simulink model "ACC4_FFNN_trainoss_30_30_30_ep_100_Nor_20250528"  (R2021a)
settings: Solver=FixedStepAuto  StartTime=0.0  StopTime=T  RelTol=1e-3
undefined symbols (not defined in the file or in its folder): t_gap, Ts, v0_ego, v0_lead, v_set, x0_ego, x0_lead, x_gain, x_offset, y_gain, y_offset
libraries: neural x95
(part 1 of 5)
settings Model: Creator=The MathWorks, Inc.  LastModifiedBy=deyun
settings SolverCC: AlgebraicLoopSolver=TrustRegion
settings DataIOCC: ReturnWorkspaceOutputs=off
settings DebuggingCC: ArithmeticOperatorsInVariantConditions=warning
settings SFSimCC: SimUseLocalCustomCode=off  CustomCodeUndefinedFunction=UseInterfaceOnly
settings RTWCC: RTWUseLocalCustomCode=off
settings CodeAppCC: StateflowObjectComments=on

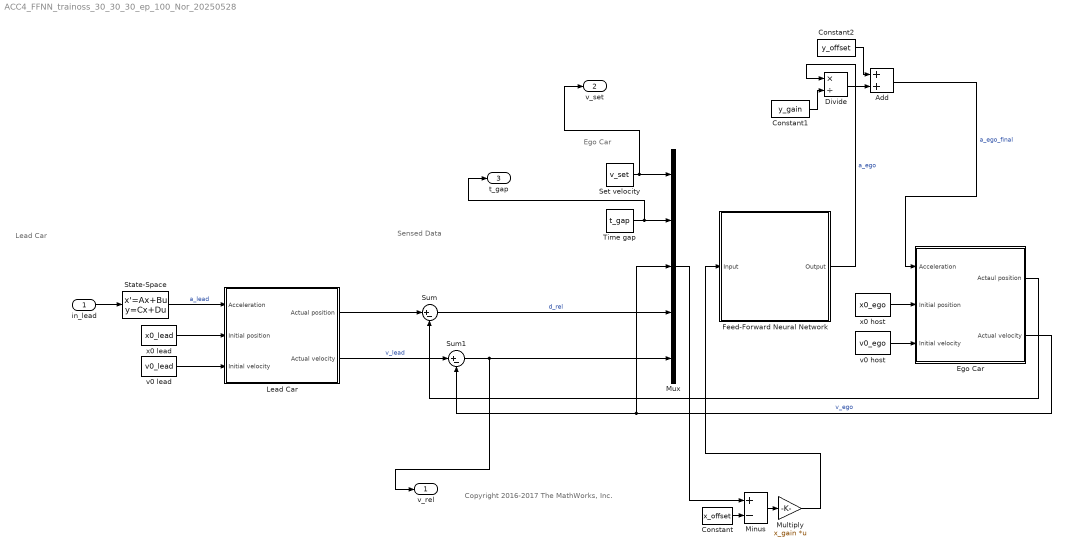
== system ACC4_FFNN_trainoss_30_30_30_ep_100_Nor_20250528 ==
  note: Sensed Data
  note: Lead Car
  note: Ego Car
  note: Copyright 2016-2017 The MathWorks, Inc.
  in_lead : Inport
  Add : Sum
  Constant : Constant  Value=x_offset
  Constant1 : Constant  Value=y_gain
  Constant2 : Constant  Value=y_offset
  Divide : Product  Inputs=*/
  Ego Car : Subsystem
  Feed-Forward Neural Network : Subsystem
      mask help: Feed-Forward Neural Network
      mask Display: e = 0.06;c1 = [120 150 230]/255;c2 = ([120 150 230]+0)/383;c3 = ([120 150 230]+128)/383;patch([0 1 1 0],[0 0 1 1],c1);patch([0 1 1 1-e 1-e 0+e],[0 0 1 1-e 0+e 0+e],c2);patch([0 0 1 1-e 0+e 0+e],[0 1 1 1-e 1-e 0+e],c3);plot([0 1 1 0 0],[0 0 1 1 0]);fprintf('NNET');port_label('input',1,' Input');port_label('output',1,'Output ');
  Lead Car : Subsystem
  Minus : Sum  Inputs=+-
  Multiply : Gain  Gain=x_gain  Multiplication=Matrix(K*u)
  Mux : Mux  Inputs=5
  Set velocity : Constant  Value=v_set  SampleTime=Ts
  State-Space : StateSpace  A=-10  B=10  D=0  InitialCondition=0
  Sum : Sum  Inputs=|+-
  Sum1 : Sum  Inputs=|+-
  Time gap : Constant  Value=t_gap  SampleTime=Ts
  v0 host : Constant  Value=v0_ego  SampleTime=Ts
  v0 lead : Constant  Value=v0_lead  SampleTime=Ts
  x0 host : Constant  Value=x0_ego  SampleTime=Ts
  x0 lead : Constant  Value=x0_lead  SampleTime=Ts
  v_rel : Outport
  v_set : Outport  Port=2
  t_gap : Outport  Port=3
  wires:
  x0 lead/1 -> Lead Car/2(Initial position)
  v0 lead/1 -> Lead Car/3(Initial velocity)
  x0 host/1 -> Ego Car/2(Initial position)
  Ego Car/1(Actaul position) -> Sum/2
  Ego Car/2(Actual velocity) -> Mux/3, Sum1/2  "v_ego"
  v0 host/1 -> Ego Car/3(Initial velocity)
  Set velocity/1 -> v_set/1, Mux/1
  Feed-Forward Neural Network/1(Output) -> Divide/1  "a_ego"
  Lead Car/1(Actual position) -> Sum/1
  Sum1/1 -> v_rel/1, Mux/5
  State-Space/1 -> Lead Car/1(Acceleration)  "a_lead"
  Lead Car/2(Actual velocity) -> Sum1/1  "v_lead"
  Sum/1 -> Mux/4  "d_rel"
  in_lead/1 -> State-Space/1
  Time gap/1 -> t_gap/1, Mux/2
  Mux/1 -> Minus/1
  Minus/1 -> Multiply/1
  Constant/1 -> Minus/2
  Multiply/1 -> Feed-Forward Neural Network/1(Input)
  Constant1/1 -> Divide/2
  Divide/1 -> Add/2
  Constant2/1 -> Add/1
  Add/1 -> Ego Car/1(Acceleration)  "a_ego_final"

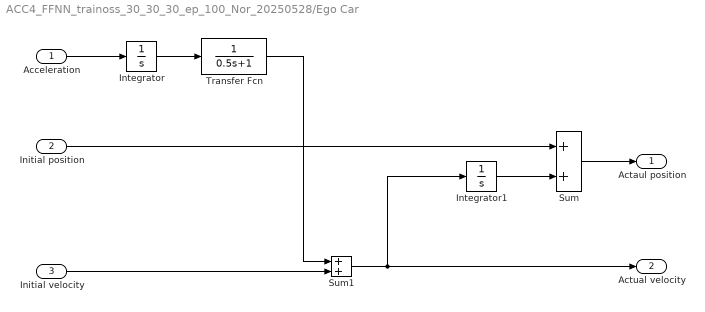
== system ACC4_FFNN_trainoss_30_30_30_ep_100_Nor_20250528/Ego Car ==
  Acceleration : Inport
  Initial position : Inport  Port=2
  Initial velocity : Inport  Port=3
  Integrator : Integrator
  Integrator1 : Integrator
  Sum : Sum
  Sum1 : Sum
  Transfer Fcn : TransferFcn  Denominator=[0.5 1]
  Actaul position : Outport  VectorParamsAs1DForOutWhenUnconnected=off
  Actual velocity : Outport  Port=2  VectorParamsAs1DForOutWhenUnconnected=off
  wires:
  Sum1/1 -> Integrator1/1, Actual velocity/1
  Initial velocity/1 -> Sum1/2
  Sum/1 -> Actaul position/1
  Transfer Fcn/1 -> Sum1/1
  Integrator/1 -> Transfer Fcn/1
  Acceleration/1 -> Integrator/1
  Initial position/1 -> Sum/1
  Integrator1/1 -> Sum/2

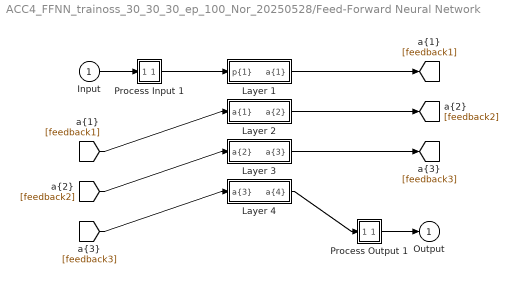
== system ACC4_FFNN_trainoss_30_30_30_ep_100_Nor_20250528/Feed-Forward Neural Network ==
  Input : Inport  PortDimensions=5
      mask Display: e = 0.06;c1 = [120 230 180]/255;c2 = ([120 230 180]+0)/(256+128);c3 = ([120 230 180]+128)/(256+128);patch([0 1 1 0],[0 0 1 1],c1);patch([0 1 1 1-e 1-e 0+e],[0 0 1 1-e 0+e 0+e],c2);patch([0 0 1 1-e 0+e 0+e],[0 1 1 1-e 1-e 0+e],c3);plot([0 1 1 0 0],[0 0 1 1 0]);
  Layer 1 : Subsystem
      mask Display: e = 0.06;c1 = [120 150 230]/255;c2 = ([120 150 230]+0)/383;c3 = ([120 150 230]+128)/383;patch([0 1 1 0],[0 0 1 1],c1);patch([0 1 1 1-e 1-e 0+e],[0 0 1 1-e 0+e 0+e],c2);patch([0 0 1 1-e 0+e 0+e],[0 1 1 1-e 1-e 0+e],c3);plot([0 1 1 0 0],[0 0 1 1 0]);
  Layer 2 : Subsystem
      mask Display: e = 0.06;c1 = [120 150 230]/255;c2 = ([120 150 230]+0)/383;c3 = ([120 150 230]+128)/383;patch([0 1 1 0],[0 0 1 1],c1);patch([0 1 1 1-e 1-e 0+e],[0 0 1 1-e 0+e 0+e],c2);patch([0 0 1 1-e 0+e 0+e],[0 1 1 1-e 1-e 0+e],c3);plot([0 1 1 0 0],[0 0 1 1 0]);
  Layer 3 : Subsystem
      mask Display: e = 0.06;c1 = [120 150 230]/255;c2 = ([120 150 230]+0)/383;c3 = ([120 150 230]+128)/383;patch([0 1 1 0],[0 0 1 1],c1);patch([0 1 1 1-e 1-e 0+e],[0 0 1 1-e 0+e 0+e],c2);patch([0 0 1 1-e 0+e 0+e],[0 1 1 1-e 1-e 0+e],c3);plot([0 1 1 0 0],[0 0 1 1 0]);
  Layer 4 : Subsystem
      mask Display: e = 0.06;c1 = [120 150 230]/255;c2 = ([120 150 230]+0)/383;c3 = ([120 150 230]+128)/383;patch([0 1 1 0],[0 0 1 1],c1);patch([0 1 1 1-e 1-e 0+e],[0 0 1 1-e 0+e 0+e],c2);patch([0 0 1 1-e 0+e 0+e],[0 1 1 1-e 1-e 0+e],c3);plot([0 1 1 0 0],[0 0 1 1 0]);
  Process Input 1 : Subsystem
      mask Display: e = 0.06;c1 = [120 150 230]/255;c2 = ([120 150 230]+0)/383;c3 = ([120 150 230]+128)/383;patch([0 1 1 0],[0 0 1 1],c1);patch([0 1 1 1-e 1-e 0+e],[0 0 1 1-e 0+e 0+e],c2);patch([0 0 1 1-e 0+e 0+e],[0 1 1 1-e 1-e 0+e],c3);plot([0 1 1 0 0],[0 0 1 1 0]);
  Process Output 1 : Subsystem
      mask Display: e = 0.06;c1 = [120 150 230]/255;c2 = ([120 150 230]+0)/383;c3 = ([120 150 230]+128)/383;patch([0 1 1 0],[0 0 1 1],c1);patch([0 1 1 1-e 1-e 0+e],[0 0 1 1-e 0+e 0+e],c2);patch([0 0 1 1-e 0+e 0+e],[0 1 1 1-e 1-e 0+e],c3);plot([0 1 1 0 0],[0 0 1 1 0]);
  Output : Outport  InitialOutput=0
      mask Display: e = 0.06;c1 = [120 230 180]/255;c2 = ([120 230 180]+0)/(256+128);c3 = ([120 230 180]+128)/(256+128);patch([0 1 1 0],[0 0 1 1],c1);patch([0 1 1 1-e 1-e 0+e],[0 0 1 1-e 0+e 0+e],c2);patch([0 0 1 1-e 0+e 0+e],[0 1 1 1-e 1-e 0+e],c3);plot([0 1 1 0 0],[0 0 1 1 0]);
  wires:
  Layer 4/1("a{4}") -> Process Output 1/1(a)
  [feedback3] -> Layer 4/1("a{3} ")
  Layer 3/1("a{3}") -> [feedback3]
  [feedback2] -> Layer 3/1("a{2} ")
  Layer 2/1("a{2}") -> [feedback2]
  [feedback1] -> Layer 2/1("a{1} ")
  Layer 1/1("a{1}") -> [feedback1]
  Process Input 1/1(p) -> Layer 1/1("p{1}")
  Process Output 1/1(y) -> Output/1
  Input/1 -> Process Input 1/1(x)

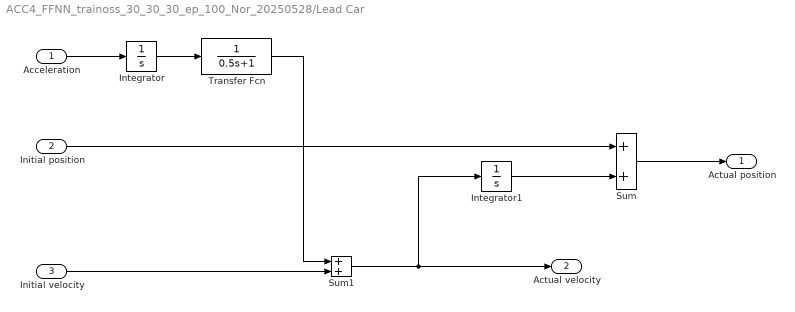
== system ACC4_FFNN_trainoss_30_30_30_ep_100_Nor_20250528/Lead Car ==
  Acceleration : Inport
  Initial position : Inport  Port=2
  Initial velocity : Inport  Port=3
  Integrator : Integrator
  Integrator1 : Integrator
  Sum : Sum
  Sum1 : Sum
  Transfer Fcn : TransferFcn  Denominator=[0.5 1]
  Actual position : Outport  VectorParamsAs1DForOutWhenUnconnected=off
  Actual velocity : Outport  Port=2  VectorParamsAs1DForOutWhenUnconnected=off
  wires:
  Transfer Fcn/1 -> Sum1/1
  Initial velocity/1 -> Sum1/2
  Sum/1 -> Actual position/1
  Integrator/1 -> Transfer Fcn/1
  Sum1/1 -> Integrator1/1, Actual velocity/1
  Acceleration/1 -> Integrator/1
  Initial position/1 -> Sum/1
  Integrator1/1 -> Sum/2

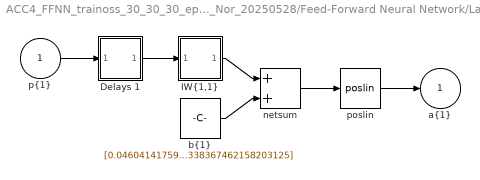
== system ACC4_FFNN_trainoss_30_30_30_ep_100_Nor_20250528/Feed-Forward Neural Network/Layer 1 ==
  "p{1}" : Inport  PortDimensions=5
      mask Display: e = 0.06;c1 = [120 230 180]/255;c2 = ([120 230 180]+0)/(256+128);c3 = ([120 230 180]+128)/(256+128);patch([0 1 1 0],[0 0 1 1],c1);patch([0 1 1 1-e 1-e 0+e],[0 0 1 1-e 0+e 0+e],c2);patch([0 0 1 1-e 0+e 0+e],[0 1 1 1-e 1-e 0+e],c3);plot([0 1 1 0 0],[0 0 1 1 0]);
  Delays 1 : Subsystem
      mask Display: e = 0.06;c1 = [120 150 230]/255;c2 = ([120 150 230]+0)/383;c3 = ([120 150 230]+128)/383;patch([0 1 1 0],[0 0 1 1],c1);patch([0 1 1 1-e 1-e 0+e],[0 0 1 1-e 0+e 0+e],c2);patch([0 0 1 1-e 0+e 0+e],[0 1 1 1-e 1-e 0+e],c3);plot([0 1 1 0 0],[0 0 1 1 0]);disp('0');
  "IW{1,1}" : Subsystem
      mask Display: e = 0.06;c1 = [120 150 230]/255;c2 = ([120 150 230]+0)/383;c3 = ([120 150 230]+128)/383;patch([0 1 1 0],[0 0 1 1],c1);patch([0 1 1 1-e 1-e 0+e],[0 0 1 1-e 0+e 0+e],c2);patch([0 0 1 1-e 0+e 0+e],[0 1 1 1-e 1-e 0+e],c3);plot([0 1 1 0 0],[0 0 1 1 0]);disp('W');
  "b{1}" : Constant  Value=[0.04604141759447825943407650584049406461417675018310546875;-0.349402015011147870637842061114497482776641845703125;0.667080116762796659912737595732323825359344482421875;0.60557904669735662661622654923121444880962371826171875;0.1282078326952769964375278277657344006001949310302734375;-0.4740719325396856032028836125391535460948944091796875;0.3611324046089003925175120457424782216548919677734375;-0.5341019862836020593022112734615802764892578125;-0.087117774565917793783142997199320234358310699462890625;-0.230866210976952146438634372316300868988037109375;0.077202877396043589897089987061917781829833984375;1.0034549741499108055364786196150816977024078369140625;0.50277941477063325947938210447318851947784423828125;0.955691922098945934038738414528779685497283935546875;-0.497741463247540483205710870606708340346813201904296875;0.04250082924725286093181608748636790551245212554931640625;-0.897127892866184328823919713613577187061309814453125;0.5137509419692445344907127946498803794384002685546875;0.20395953255102039491930554504506289958953857421875;0.70482076515493818913427048755693249404430389404296875;0.95254607457197948416904864643584005534648895263671875;0.8512508612841169775009575459989719092845916748046875;-0.1655257909270722027628153227851726114749908447265625;-1.001197592605171049484624745673500001430511474609375;0.08635824799345669100514299998394562862813472747802734375;-0.5845387560078811883812477390165440738201141357421875;-0.5614328236351393552894251115503720939159393310546875;-0.35187840556543503733877287231734953820705413818359375;-0.80810116678483101537722177454270422458648681640625;0.4950673234766060915035268408246338367462158203125]
      mask Display: e = 0.06;c1 = [120 150 230]/255;c2 = ([120 150 230]+0)/383;c3 = ([120 150 230]+128)/383;patch([0 1 1 0],[0 0 1 1],c1);patch([0 1 1 1-e 1-e 0+e],[0 0 1 1-e 0+e 0+e],c2);patch([0 0 1 1-e 0+e 0+e],[0 1 1 1-e 1-e 0+e],c3);plot([0 1 1 0 0],[0 0 1 1 0]);disp('b');
  netsum : Sum  Inputs=2  InputSameDT=on  SaturateOnIntegerOverflow=on  OutDataTypeStr=Inherit: Same as first input
      mask Display: e = 0.06;c1 = [120 150 230]/255;c2 = ([120 150 230]+0)/383;c3 = ([120 150 230]+128)/383;patch([0 1 1 0],[0 0 1 1],c1);patch([0 1 1 1-e 1-e 0+e],[0 0 1 1-e 0+e 0+e],c2);patch([0 0 1 1-e 0+e 0+e],[0 1 1 1-e 1-e 0+e],c3);plot([0 1 1 0 0],[0 0 1 1 0]);disp('+');
  poslin : neural/Transfer Functions/poslin
      settings: SourceProductBaseCode=NN
  "a{1}" : Outport  InitialOutput=[0;0;0;0;0;0;0;0;0;0;0;0;0;0;0;0;0;0;0;0;0;0;0;0;0;0;0;0;0;0]
      mask Display: e = 0.06;c1 = [120 230 180]/255;c2 = ([120 230 180]+0)/(256+128);c3 = ([120 230 180]+128)/(256+128);patch([0 1 1 0],[0 0 1 1],c1);patch([0 1 1 1-e 1-e 0+e],[0 0 1 1-e 0+e 0+e],c2);patch([0 0 1 1-e 0+e 0+e],[0 1 1 1-e 1-e 0+e],c3);plot([0 1 1 0 0],[0 0 1 1 0]);
  wires:
  poslin/1 -> "a{1}"/1
  netsum/1 -> poslin/1
  "b{1}"/1 -> netsum/2
  "IW{1,1}"/1("iz{1,1}") -> netsum/1
  Delays 1/1("pd{1,1}") -> "IW{1,1}"/1("pd{1,1}")
  "p{1}"/1 -> Delays 1/1("p{1}")

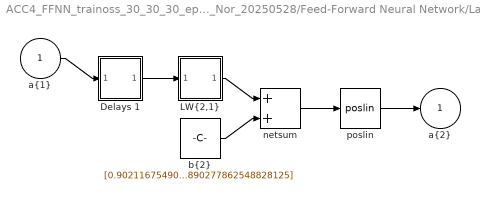
== system ACC4_FFNN_trainoss_30_30_30_ep_100_Nor_20250528/Feed-Forward Neural Network/Layer 2 ==
  "a{1} " : Inport  PortDimensions=30
      mask Display: e = 0.06;c1 = [120 230 180]/255;c2 = ([120 230 180]+0)/(256+128);c3 = ([120 230 180]+128)/(256+128);patch([0 1 1 0],[0 0 1 1],c1);patch([0 1 1 1-e 1-e 0+e],[0 0 1 1-e 0+e 0+e],c2);patch([0 0 1 1-e 0+e 0+e],[0 1 1 1-e 1-e 0+e],c3);plot([0 1 1 0 0],[0 0 1 1 0]);
  Delays 1 : Subsystem
      mask Display: e = 0.06;c1 = [120 150 230]/255;c2 = ([120 150 230]+0)/383;c3 = ([120 150 230]+128)/383;patch([0 1 1 0],[0 0 1 1],c1);patch([0 1 1 1-e 1-e 0+e],[0 0 1 1-e 0+e 0+e],c2);patch([0 0 1 1-e 0+e 0+e],[0 1 1 1-e 1-e 0+e],c3);plot([0 1 1 0 0],[0 0 1 1 0]);disp('0');
  "LW{2,1}" : Subsystem
      mask Display: e = 0.06;c1 = [120 150 230]/255;c2 = ([120 150 230]+0)/383;c3 = ([120 150 230]+128)/383;patch([0 1 1 0],[0 0 1 1],c1);patch([0 1 1 1-e 1-e 0+e],[0 0 1 1-e 0+e 0+e],c2);patch([0 0 1 1-e 0+e 0+e],[0 1 1 1-e 1-e 0+e],c3);plot([0 1 1 0 0],[0 0 1 1 0]);disp('W');
  "b{2}" : Constant  Value=[0.90211675490508869135197755895205773413181304931640625;0.96364395097861355043988851321046240627765655517578125;-0.93801236425877643210213818747433833777904510498046875;-0.01526552283014774580305328299800748936831951141357421875;0.725444256277659516030098529881797730922698974609375;-0.51151540170335441093385497879353351891040802001953125;0.66538113127496512078096202458254992961883544921875;0.6269149410732415272917705806321464478969573974609375;0.258930692402123241446787460517953149974346160888671875;-0.99391093407740893628243838975322432816028594970703125;-0.2405521205461311762263676428119651973247528076171875;0.8088428445387572107705409507616423070430755615234375;0.364640259893649842926066639847704209387302398681640625;-0.243645218450386613628921850249753333628177642822265625;0.2639094214046682207452931834268383681774139404296875;-0.5134609550588200566068053376511670649051666259765625;0.1373606272949773610125845380025566555559635162353515625;0.97668827905990884818976383030530996620655059814453125;0.69526590032446000666510599330649711191654205322265625;-0.434971195316202818847983735395246185362339019775390625;0.364915328900436097825377146364189684391021728515625;-0.279865051883634141649537241391954012215137481689453125;0.97740122180252420047708028505439870059490203857421875;-0.832027408487622466282118693925440311431884765625;-0.49423259242849260086671847602701745927333831787109375;0.626024890630703101379594954778440296649932861328125;-0.8310643492461855519337632358656264841556549072265625;0.0627983927541861941534762081573717296123504638671875;0.601245958295900440049308599554933607578277587890625;0.477951473350415156904347213639994151890277862548828125]
      mask Display: e = 0.06;c1 = [120 150 230]/255;c2 = ([120 150 230]+0)/383;c3 = ([120 150 230]+128)/383;patch([0 1 1 0],[0 0 1 1],c1);patch([0 1 1 1-e 1-e 0+e],[0 0 1 1-e 0+e 0+e],c2);patch([0 0 1 1-e 0+e 0+e],[0 1 1 1-e 1-e 0+e],c3);plot([0 1 1 0 0],[0 0 1 1 0]);disp('b');
  netsum : Sum  Inputs=2  InputSameDT=on  SaturateOnIntegerOverflow=on  OutDataTypeStr=Inherit: Same as first input
      mask Display: e = 0.06;c1 = [120 150 230]/255;c2 = ([120 150 230]+0)/383;c3 = ([120 150 230]+128)/383;patch([0 1 1 0],[0 0 1 1],c1);patch([0 1 1 1-e 1-e 0+e],[0 0 1 1-e 0+e 0+e],c2);patch([0 0 1 1-e 0+e 0+e],[0 1 1 1-e 1-e 0+e],c3);plot([0 1 1 0 0],[0 0 1 1 0]);disp('+');
  poslin : neural/Transfer Functions/poslin
      settings: SourceProductBaseCode=NN
  "a{2}" : Outport  InitialOutput=[0;0;0;0;0;0;0;0;0;0;0;0;0;0;0;0;0;0;0;0;0;0;0;0;0;0;0;0;0;0]
      mask Display: e = 0.06;c1 = [120 230 180]/255;c2 = ([120 230 180]+0)/(256+128);c3 = ([120 230 180]+128)/(256+128);patch([0 1 1 0],[0 0 1 1],c1);patch([0 1 1 1-e 1-e 0+e],[0 0 1 1-e 0+e 0+e],c2);patch([0 0 1 1-e 0+e 0+e],[0 1 1 1-e 1-e 0+e],c3);plot([0 1 1 0 0],[0 0 1 1 0]);
  wires:
  poslin/1 -> "a{2}"/1
  netsum/1 -> poslin/1
  "b{2}"/1 -> netsum/2
  "LW{2,1}"/1("lz{2,1}") -> netsum/1
  Delays 1/1("pd{2,1}") -> "LW{2,1}"/1("ad{2,1}")
  "a{1} "/1 -> Delays 1/1("p{2}")

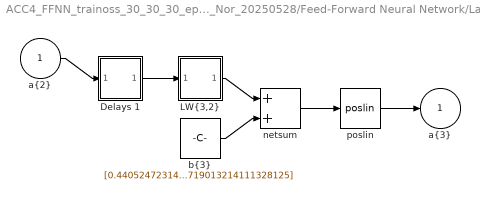
== system ACC4_FFNN_trainoss_30_30_30_ep_100_Nor_20250528/Feed-Forward Neural Network/Layer 3 ==
  "a{2} " : Inport  PortDimensions=30
      mask Display: e = 0.06;c1 = [120 230 180]/255;c2 = ([120 230 180]+0)/(256+128);c3 = ([120 230 180]+128)/(256+128);patch([0 1 1 0],[0 0 1 1],c1);patch([0 1 1 1-e 1-e 0+e],[0 0 1 1-e 0+e 0+e],c2);patch([0 0 1 1-e 0+e 0+e],[0 1 1 1-e 1-e 0+e],c3);plot([0 1 1 0 0],[0 0 1 1 0]);
  Delays 1 : Subsystem
      mask Display: e = 0.06;c1 = [120 150 230]/255;c2 = ([120 150 230]+0)/383;c3 = ([120 150 230]+128)/383;patch([0 1 1 0],[0 0 1 1],c1);patch([0 1 1 1-e 1-e 0+e],[0 0 1 1-e 0+e 0+e],c2);patch([0 0 1 1-e 0+e 0+e],[0 1 1 1-e 1-e 0+e],c3);plot([0 1 1 0 0],[0 0 1 1 0]);disp('0');
  "LW{3,2}" : Subsystem
      mask Display: e = 0.06;c1 = [120 150 230]/255;c2 = ([120 150 230]+0)/383;c3 = ([120 150 230]+128)/383;patch([0 1 1 0],[0 0 1 1],c1);patch([0 1 1 1-e 1-e 0+e],[0 0 1 1-e 0+e 0+e],c2);patch([0 0 1 1-e 0+e 0+e],[0 1 1 1-e 1-e 0+e],c3);plot([0 1 1 0 0],[0 0 1 1 0]);disp('W');
  "b{3}" : Constant  Value=[0.4405247231410467367851424569380469620227813720703125;0.357876687390491110551948850115877576172351837158203125;-0.574481979793593833250042735016904771327972412109375;-0.837153308541852769764091135584749281406402587890625;-0.45146469146650824999511542046093381941318511962890625;0.73604643553605664241246131496154703199863433837890625;0.11830618425636067747586110954216565005481243133544921875;-0.0710728139228912481062394590480835177004337310791015625;-0.1393981984391927664290733446250669658184051513671875;0.54797184004082755137687854585237801074981689453125;0.308241831903243002077630308122024871408939361572265625;0.31545304820107766818892969240550883114337921142578125;-0.67808294548384340227897837394266389310359954833984375;-0.135258081328783585917108212015591561794281005859375;0.010172168711043649835801261360757052898406982421875;-0.25362159832491959488010024870163761079311370849609375;-0.039723153024012018696975445664065773598849773406982421875;-0.31521694315790338425387062670779414474964141845703125;0.55514550915098548333759254092001356184482574462890625;-0.2321122752203861328013090314925648272037506103515625;0.42332375192715809841814689207240007817745208740234375;-0.040123747740405980855005196872298256494104862213134765625;0.45836044424314348333382440614514052867889404296875;0.8749288536162034279897170563344843685626983642578125;0.034051484090962598483276480010317754931747913360595703125;0.80611753338239744426374500108067877590656280517578125;-0.56333564819738002338311844141571782529354095458984375;0.746490829761710994461054724524728953838348388671875;-0.8343950519130831633418665660428814589977264404296875;-0.06910200297563613702767071345078875310719013214111328125]
      mask Display: e = 0.06;c1 = [120 150 230]/255;c2 = ([120 150 230]+0)/383;c3 = ([120 150 230]+128)/383;patch([0 1 1 0],[0 0 1 1],c1);patch([0 1 1 1-e 1-e 0+e],[0 0 1 1-e 0+e 0+e],c2);patch([0 0 1 1-e 0+e 0+e],[0 1 1 1-e 1-e 0+e],c3);plot([0 1 1 0 0],[0 0 1 1 0]);disp('b');
  netsum : Sum  Inputs=2  InputSameDT=on  SaturateOnIntegerOverflow=on  OutDataTypeStr=Inherit: Same as first input
      mask Display: e = 0.06;c1 = [120 150 230]/255;c2 = ([120 150 230]+0)/383;c3 = ([120 150 230]+128)/383;patch([0 1 1 0],[0 0 1 1],c1);patch([0 1 1 1-e 1-e 0+e],[0 0 1 1-e 0+e 0+e],c2);patch([0 0 1 1-e 0+e 0+e],[0 1 1 1-e 1-e 0+e],c3);plot([0 1 1 0 0],[0 0 1 1 0]);disp('+');
  poslin : neural/Transfer Functions/poslin
      settings: SourceProductBaseCode=NN
  "a{3}" : Outport  InitialOutput=[0;0;0;0;0;0;0;0;0;0;0;0;0;0;0;0;0;0;0;0;0;0;0;0;0;0;0;0;0;0]
      mask Display: e = 0.06;c1 = [120 230 180]/255;c2 = ([120 230 180]+0)/(256+128);c3 = ([120 230 180]+128)/(256+128);patch([0 1 1 0],[0 0 1 1],c1);patch([0 1 1 1-e 1-e 0+e],[0 0 1 1-e 0+e 0+e],c2);patch([0 0 1 1-e 0+e 0+e],[0 1 1 1-e 1-e 0+e],c3);plot([0 1 1 0 0],[0 0 1 1 0]);
  wires:
  poslin/1 -> "a{3}"/1
  netsum/1 -> poslin/1
  "b{3}"/1 -> netsum/2
  "LW{3,2}"/1("lz{3,2}") -> netsum/1
  Delays 1/1("pd{3,2}") -> "LW{3,2}"/1("ad{3,2}")
  "a{2} "/1 -> Delays 1/1("p{3}")

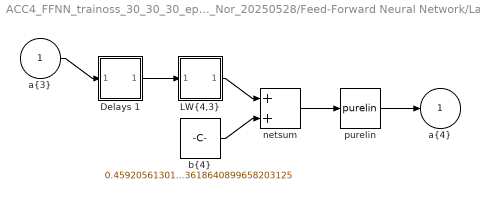
== system ACC4_FFNN_trainoss_30_30_30_ep_100_Nor_20250528/Feed-Forward Neural Network/Layer 4 ==
  "a{3} " : Inport  PortDimensions=30
      mask Display: e = 0.06;c1 = [120 230 180]/255;c2 = ([120 230 180]+0)/(256+128);c3 = ([120 230 180]+128)/(256+128);patch([0 1 1 0],[0 0 1 1],c1);patch([0 1 1 1-e 1-e 0+e],[0 0 1 1-e 0+e 0+e],c2);patch([0 0 1 1-e 0+e 0+e],[0 1 1 1-e 1-e 0+e],c3);plot([0 1 1 0 0],[0 0 1 1 0]);
  Delays 1 : Subsystem
      mask Display: e = 0.06;c1 = [120 150 230]/255;c2 = ([120 150 230]+0)/383;c3 = ([120 150 230]+128)/383;patch([0 1 1 0],[0 0 1 1],c1);patch([0 1 1 1-e 1-e 0+e],[0 0 1 1-e 0+e 0+e],c2);patch([0 0 1 1-e 0+e 0+e],[0 1 1 1-e 1-e 0+e],c3);plot([0 1 1 0 0],[0 0 1 1 0]);disp('0');
  "LW{4,3}" : Subsystem
      mask Display: e = 0.06;c1 = [120 150 230]/255;c2 = ([120 150 230]+0)/383;c3 = ([120 150 230]+128)/383;patch([0 1 1 0],[0 0 1 1],c1);patch([0 1 1 1-e 1-e 0+e],[0 0 1 1-e 0+e 0+e],c2);patch([0 0 1 1-e 0+e 0+e],[0 1 1 1-e 1-e 0+e],c3);plot([0 1 1 0 0],[0 0 1 1 0]);disp('W');
  "b{4}" : Constant  Value=0.459205613013363933561095109325833618640899658203125
      mask Display: e = 0.06;c1 = [120 150 230]/255;c2 = ([120 150 230]+0)/383;c3 = ([120 150 230]+128)/383;patch([0 1 1 0],[0 0 1 1],c1);patch([0 1 1 1-e 1-e 0+e],[0 0 1 1-e 0+e 0+e],c2);patch([0 0 1 1-e 0+e 0+e],[0 1 1 1-e 1-e 0+e],c3);plot([0 1 1 0 0],[0 0 1 1 0]);disp('b');
  netsum : Sum  Inputs=2  InputSameDT=on  SaturateOnIntegerOverflow=on  OutDataTypeStr=Inherit: Same as first input
      mask Display: e = 0.06;c1 = [120 150 230]/255;c2 = ([120 150 230]+0)/383;c3 = ([120 150 230]+128)/383;patch([0 1 1 0],[0 0 1 1],c1);patch([0 1 1 1-e 1-e 0+e],[0 0 1 1-e 0+e 0+e],c2);patch([0 0 1 1-e 0+e 0+e],[0 1 1 1-e 1-e 0+e],c3);plot([0 1 1 0 0],[0 0 1 1 0]);disp('+');
  purelin : neural/Transfer Functions/purelin
  "a{4}" : Outport  InitialOutput=0
      mask Display: e = 0.06;c1 = [120 230 180]/255;c2 = ([120 230 180]+0)/(256+128);c3 = ([120 230 180]+128)/(256+128);patch([0 1 1 0],[0 0 1 1],c1);patch([0 1 1 1-e 1-e 0+e],[0 0 1 1-e 0+e 0+e],c2);patch([0 0 1 1-e 0+e 0+e],[0 1 1 1-e 1-e 0+e],c3);plot([0 1 1 0 0],[0 0 1 1 0]);
  wires:
  purelin/1 -> "a{4}"/1
  netsum/1 -> purelin/1
  "b{4}"/1 -> netsum/2
  "LW{4,3}"/1("lz{4,3}") -> netsum/1
  Delays 1/1("pd{4,3}") -> "LW{4,3}"/1("ad{4,3}")
  "a{3} "/1 -> Delays 1/1("p{4}")

== system ACC4_FFNN_trainoss_30_30_30_ep_100_Nor_20250528/Feed-Forward Neural Network/Process Input 1 ==
  x : Inport  PortDimensions=5
      mask Display: e = 0.06;c1 = [120 230 180]/255;c2 = ([120 230 180]+0)/(256+128);c3 = ([120 230 180]+128)/(256+128);patch([0 1 1 0],[0 0 1 1],c1);patch([0 1 1 1-e 1-e 0+e],[0 0 1 1-e 0+e 0+e],c2);patch([0 0 1 1-e 0+e 0+e],[0 1 1 1-e 1-e 0+e],c3);plot([0 1 1 0 0],[0 0 1 1 0]);
  p : Outport  PortDimensions=5
      mask Display: e = 0.06;c1 = [120 230 180]/255;c2 = ([120 230 180]+0)/(256+128);c3 = ([120 230 180]+128)/(256+128);patch([0 1 1 0],[0 0 1 1],c1);patch([0 1 1 1-e 1-e 0+e],[0 0 1 1-e 0+e 0+e],c2);patch([0 0 1 1-e 0+e 0+e],[0 1 1 1-e 1-e 0+e],c3);plot([0 1 1 0 0],[0 0 1 1 0]);
  wires:
  x/1 -> p/1

== system ACC4_FFNN_trainoss_30_30_30_ep_100_Nor_20250528/Feed-Forward Neural Network/Process Output 1 ==
  a : Inport  PortDimensions=1
      mask Display: e = 0.06;c1 = [120 230 180]/255;c2 = ([120 230 180]+0)/(256+128);c3 = ([120 230 180]+128)/(256+128);patch([0 1 1 0],[0 0 1 1],c1);patch([0 1 1 1-e 1-e 0+e],[0 0 1 1-e 0+e 0+e],c2);patch([0 0 1 1-e 0+e 0+e],[0 1 1 1-e 1-e 0+e],c3);plot([0 1 1 0 0],[0 0 1 1 0]);
  y : Outport  PortDimensions=1
      mask Display: e = 0.06;c1 = [120 230 180]/255;c2 = ([120 230 180]+0)/(256+128);c3 = ([120 230 180]+128)/(256+128);patch([0 1 1 0],[0 0 1 1],c1);patch([0 1 1 1-e 1-e 0+e],[0 0 1 1-e 0+e 0+e],c2);patch([0 0 1 1-e 0+e 0+e],[0 1 1 1-e 1-e 0+e],c3);plot([0 1 1 0 0],[0 0 1 1 0]);
  wires:
  a/1 -> y/1

== system ACC4_FFNN_trainoss_30_30_30_ep_100_Nor_20250528/Feed-Forward Neural Network/Layer 1/Delays 1 ==
  "p{1}" : Inport  PortDimensions=5
      mask Display: e = 0.06;c1 = [120 230 180]/255;c2 = ([120 230 180]+0)/(256+128);c3 = ([120 230 180]+128)/(256+128);patch([0 1 1 0],[0 0 1 1],c1);patch([0 1 1 1-e 1-e 0+e],[0 0 1 1-e 0+e 0+e],c2);patch([0 0 1 1-e 0+e 0+e],[0 1 1 1-e 1-e 0+e],c3);plot([0 1 1 0 0],[0 0 1 1 0]);
  mux : Mux  Inputs=1
      mask Display: e = 0.06;c1 = [120 150 230]/255;c2 = ([120 150 230]+0)/383;c3 = ([120 150 230]+128)/383;patch([0 1 1 0],[0 0 1 1],c1);patch([0 1 1 1-e 1-e 0+e],[0 0 1 1-e 0+e 0+e],c2);patch([0 0 1 1-e 0+e 0+e],[0 1 1 1-e 1-e 0+e],c3);plot([0 1 1 0 0],[0 0 1 1 0]);disp('Mux')
  "pd{1,1}" : Outport
      mask Display: e = 0.06;c1 = [120 230 180]/255;c2 = ([120 230 180]+0)/(256+128);c3 = ([120 230 180]+128)/(256+128);patch([0 1 1 0],[0 0 1 1],c1);patch([0 1 1 1-e 1-e 0+e],[0 0 1 1-e 0+e 0+e],c2);patch([0 0 1 1-e 0+e 0+e],[0 1 1 1-e 1-e 0+e],c3);plot([0 1 1 0 0],[0 0 1 1 0]);
  wires:
  mux/1 -> "pd{1,1}"/1
  "p{1}"/1 -> mux/1

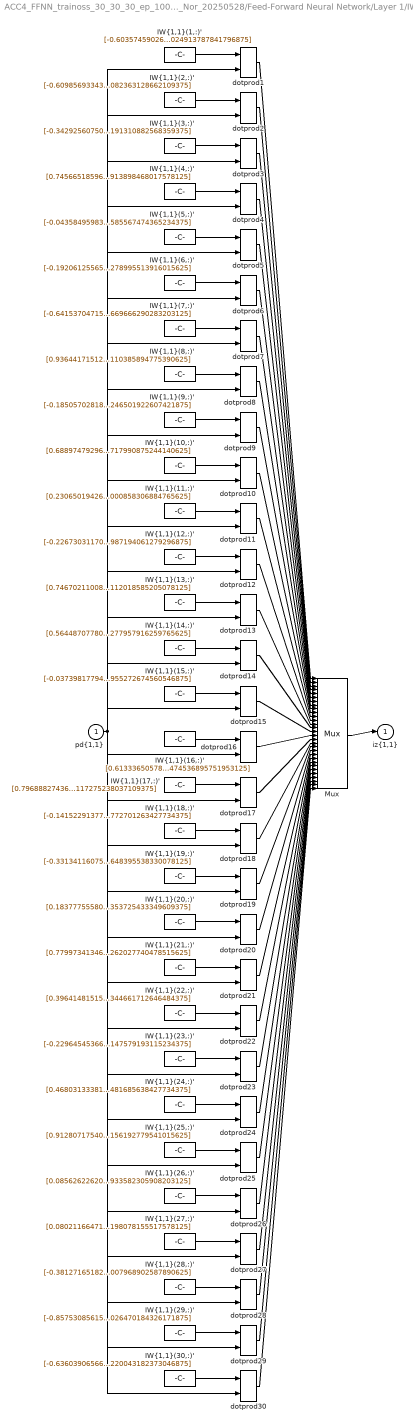
== system ACC4_FFNN_trainoss_30_30_30_ep_100_Nor_20250528/Feed-Forward Neural Network/Layer 1/IW{1,1} ==
  "pd{1,1}" : Inport  PortDimensions=5
      mask Display: e = 0.06;c1 = [120 230 180]/255;c2 = ([120 230 180]+0)/(256+128);c3 = ([120 230 180]+128)/(256+128);patch([0 1 1 0],[0 0 1 1],c1);patch([0 1 1 1-e 1-e 0+e],[0 0 1 1-e 0+e 0+e],c2);patch([0 0 1 1-e 0+e 0+e],[0 1 1 1-e 1-e 0+e],c3);plot([0 1 1 0 0],[0 0 1 1 0]);
  "IW{1,1}(1,:)'" : Constant  Value=[-0.6035745902618299130182322187465615570545196533203125;-0.814040325548151866286161748575977981090545654296875;-0.0775546564559805029492878247765474952757358551025390625;0.713774809937765208900373181677423417568206787109375;0.7908289690471679289629491904634051024913787841796875]
      mask Display: e = 0.06;c1 = [120 150 230]/255;c2 = ([120 150 230]+0)/383;c3 = ([120 150 230]+128)/383;patch([0 1 1 0],[0 0 1 1],c1);patch([0 1 1 1-e 1-e 0+e],[0 0 1 1-e 0+e 0+e],c2);patch([0 0 1 1-e 0+e 0+e],[0 1 1 1-e 1-e 0+e],c3);plot([0 1 1 0 0],[0 0 1 1 0]);disp('Weights');
  "IW{1,1}(10,:)'" : Constant  Value=[0.6889747929668963433158523912425152957439422607421875;-0.745467933349733158365779672749340534210205078125;-0.64204969474453577049644081853330135345458984375;0.799965592865721664139755375799722969532012939453125;-0.6903424584977886357961551766493357717990875244140625]
      mask Display: e = 0.06;c1 = [120 150 230]/255;c2 = ([120 150 230]+0)/383;c3 = ([120 150 230]+128)/383;patch([0 1 1 0],[0 0 1 1],c1);patch([0 1 1 1-e 1-e 0+e],[0 0 1 1-e 0+e 0+e],c2);patch([0 0 1 1-e 0+e 0+e],[0 1 1 1-e 1-e 0+e],c3);plot([0 1 1 0 0],[0 0 1 1 0]);disp('Weights');
  "IW{1,1}(11,:)'" : Constant  Value=[0.230650194261698970876750536262989044189453125;-0.982704624243819324647120083682239055633544921875;0.2666671606402430949600557141820900142192840576171875;-0.6131324961218160840559221469447948038578033447265625;-0.71218334265026417284616400138475000858306884765625]
      mask Display: e = 0.06;c1 = [120 150 230]/255;c2 = ([120 150 230]+0)/383;c3 = ([120 150 230]+128)/383;patch([0 1 1 0],[0 0 1 1],c1);patch([0 1 1 1-e 1-e 0+e],[0 0 1 1-e 0+e 0+e],c2);patch([0 0 1 1-e 0+e 0+e],[0 1 1 1-e 1-e 0+e],c3);plot([0 1 1 0 0],[0 0 1 1 0]);disp('Weights');
  "IW{1,1}(12,:)'" : Constant  Value=[-0.2267303117085231745075901699237874709069728851318359375;0.474206734523056783192629382028826512396335601806640625;0.26408373958160080707813222034019418060779571533203125;0.500370970455730645909397935611195862293243408203125;0.2109635849565252019299776975458371452987194061279296875]
      mask Display: e = 0.06;c1 = [120 150 230]/255;c2 = ([120 150 230]+0)/383;c3 = ([120 150 230]+128)/383;patch([0 1 1 0],[0 0 1 1],c1);patch([0 1 1 1-e 1-e 0+e],[0 0 1 1-e 0+e 0+e],c2);patch([0 0 1 1-e 0+e 0+e],[0 1 1 1-e 1-e 0+e],c3);plot([0 1 1 0 0],[0 0 1 1 0]);disp('Weights');
  "IW{1,1}(13,:)'" : Constant  Value=[0.7467021100891664264764813196961767971515655517578125;-0.2994284564718541208350188753684051334857940673828125;-0.34647222778537012377597648082883097231388092041015625;-0.301149598852876565491243354699690826237201690673828125;-0.48712599542628531867904939645086415112018585205078125]
      mask Display: e = 0.06;c1 = [120 150 230]/255;c2 = ([120 150 230]+0)/383;c3 = ([120 150 230]+128)/383;patch([0 1 1 0],[0 0 1 1],c1);patch([0 1 1 1-e 1-e 0+e],[0 0 1 1-e 0+e 0+e],c2);patch([0 0 1 1-e 0+e 0+e],[0 1 1 1-e 1-e 0+e],c3);plot([0 1 1 0 0],[0 0 1 1 0]);disp('Weights');
  "IW{1,1}(14,:)'" : Constant  Value=[0.56448707780424489666160070555633865296840667724609375;0.55567411543024680664615289060748182237148284912109375;0.6064682491764650240639866751735098659992218017578125;-0.164601177501819073700772833035443909466266632080078125;-0.350865032772584461984166637193993665277957916259765625]
      mask Display: e = 0.06;c1 = [120 150 230]/255;c2 = ([120 150 230]+0)/383;c3 = ([120 150 230]+128)/383;patch([0 1 1 0],[0 0 1 1],c1);patch([0 1 1 1-e 1-e 0+e],[0 0 1 1-e 0+e 0+e],c2);patch([0 0 1 1-e 0+e 0+e],[0 1 1 1-e 1-e 0+e],c3);plot([0 1 1 0 0],[0 0 1 1 0]);disp('Weights');
  "IW{1,1}(15,:)'" : Constant  Value=[-0.037398177944166173525264440513637964613735675811767578125;-0.09399346130265238963286122952922596596181392669677734375;1.03004059637241329738799322512932121753692626953125;-0.702219974967766003004498998052440583705902099609375;-0.187530076933664968663606487098149955272674560546875]
      mask Display: e = 0.06;c1 = [120 150 230]/255;c2 = ([120 150 230]+0)/383;c3 = ([120 150 230]+128)/383;patch([0 1 1 0],[0 0 1 1],c1);patch([0 1 1 1-e 1-e 0+e],[0 0 1 1-e 0+e 0+e],c2);patch([0 0 1 1-e 0+e 0+e],[0 1 1 1-e 1-e 0+e],c3);plot([0 1 1 0 0],[0 0 1 1 0]);disp('Weights');
  "IW{1,1}(16,:)'" : Constant  Value=[0.61333650578379017570540554515901021659374237060546875;-0.1415077831135414243579617732393671758472919464111328125;0.95259759144218347781674083307734690606594085693359375;0.61944232418416589336374045160482637584209442138671875;-0.19945544925436398120410785850253887474536895751953125]
      mask Display: e = 0.06;c1 = [120 150 230]/255;c2 = ([120 150 230]+0)/383;c3 = ([120 150 230]+128)/383;patch([0 1 1 0],[0 0 1 1],c1);patch([0 1 1 1-e 1-e 0+e],[0 0 1 1-e 0+e 0+e],c2);patch([0 0 1 1-e 0+e 0+e],[0 1 1 1-e 1-e 0+e],c3);plot([0 1 1 0 0],[0 0 1 1 0]);disp('Weights');
  "IW{1,1}(17,:)'" : Constant  Value=[0.796888274360240789206955014378763735294342041015625;-0.901573639287027273070407318300567567348480224609375;-0.7459261156102858780769793156650848686695098876953125;0.24984705569255449830734505667351186275482177734375;-0.2276177228781752770458979284740053117275238037109375]
      mask Display: e = 0.06;c1 = [120 150 230]/255;c2 = ([120 150 230]+0)/383;c3 = ([120 150 230]+128)/383;patch([0 1 1 0],[0 0 1 1],c1);patch([0 1 1 1-e 1-e 0+e],[0 0 1 1-e 0+e 0+e],c2);patch([0 0 1 1-e 0+e 0+e],[0 1 1 1-e 1-e 0+e],c3);plot([0 1 1 0 0],[0 0 1 1 0]);disp('Weights');
  "IW{1,1}(18,:)'" : Constant  Value=[-0.141522913770345315498389027197845280170440673828125;-0.900736196961219537371334808995015919208526611328125;-0.535519708076414691078070973162539303302764892578125;0.4771208432212954431150819800677709281444549560546875;0.21960364767590956347476094379089772701263427734375]
      mask Display: e = 0.06;c1 = [120 150 230]/255;c2 = ([120 150 230]+0)/383;c3 = ([120 150 230]+128)/383;patch([0 1 1 0],[0 0 1 1],c1);patch([0 1 1 1-e 1-e 0+e],[0 0 1 1-e 0+e 0+e],c2);patch([0 0 1 1-e 0+e 0+e],[0 1 1 1-e 1-e 0+e],c3);plot([0 1 1 0 0],[0 0 1 1 0]);disp('Weights');
  "IW{1,1}(19,:)'" : Constant  Value=[-0.331341160755560526496310558286495506763458251953125;-0.8177996491738921402969708651653490960597991943359375;-0.9527350666835499026774414232932031154632568359375;0.6102248414139079812912314082495868206024169921875;-0.6662185546675083447354381860350258648395538330078125]
      mask Display: e = 0.06;c1 = [120 150 230]/255;c2 = ([120 150 230]+0)/383;c3 = ([120 150 230]+128)/383;patch([0 1 1 0],[0 0 1 1],c1);patch([0 1 1 1-e 1-e 0+e],[0 0 1 1-e 0+e 0+e],c2);patch([0 0 1 1-e 0+e 0+e],[0 1 1 1-e 1-e 0+e],c3);plot([0 1 1 0 0],[0 0 1 1 0]);disp('Weights');
  "IW{1,1}(2,:)'" : Constant  Value=[-0.6098569334314782874884031116380356252193450927734375;-0.07302150447551358780629016109742224216461181640625;0.278647524398712764792662710533477365970611572265625;-0.9132190568660936147438178522861562669277191162109375;0.1650370493360602264232284142053686082363128662109375]
      mask Display: e = 0.06;c1 = [120 150 230]/255;c2 = ([120 150 230]+0)/383;c3 = ([120 150 230]+128)/383;patch([0 1 1 0],[0 0 1 1],c1);patch([0 1 1 1-e 1-e 0+e],[0 0 1 1-e 0+e 0+e],c2);patch([0 0 1 1-e 0+e 0+e],[0 1 1 1-e 1-e 0+e],c3);plot([0 1 1 0 0],[0 0 1 1 0]);disp('Weights');
  "IW{1,1}(20,:)'" : Constant  Value=[0.1837775558010134313580152820577495731413364410400390625;0.1785574097987633612749647227246896363794803619384765625;0.2030505269833618176011924560953048057854175567626953125;-0.858854418630413452007132946164347231388092041015625;-0.623797073242660982117513412958942353725433349609375]
      mask Display: e = 0.06;c1 = [120 150 230]/255;c2 = ([120 150 230]+0)/383;c3 = ([120 150 230]+128)/383;patch([0 1 1 0],[0 0 1 1],c1);patch([0 1 1 1-e 1-e 0+e],[0 0 1 1-e 0+e 0+e],c2);patch([0 0 1 1-e 0+e 0+e],[0 1 1 1-e 1-e 0+e],c3);plot([0 1 1 0 0],[0 0 1 1 0]);disp('Weights');
  "IW{1,1}(21,:)'" : Constant  Value=[0.7799734134688771636234605466597713530063629150390625;-0.541840093606202888310008347616530954837799072265625;-0.7912594232903911173337974105379544198513031005859375;0.87721976491920672369673184221028350293636322021484375;-0.827351363023736130486440742970444262027740478515625]
      mask Display: e = 0.06;c1 = [120 150 230]/255;c2 = ([120 150 230]+0)/383;c3 = ([120 150 230]+128)/383;patch([0 1 1 0],[0 0 1 1],c1);patch([0 1 1 1-e 1-e 0+e],[0 0 1 1-e 0+e 0+e],c2);patch([0 0 1 1-e 0+e 0+e],[0 1 1 1-e 1-e 0+e],c3);plot([0 1 1 0 0],[0 0 1 1 0]);disp('Weights');
  "IW{1,1}(22,:)'" : Constant  Value=[0.3964148151522344232233763250405900180339813232421875;0.67502012037717040726647610426880419254302978515625;-0.185910849422085633353418643309851177036762237548828125;-0.01395566199154268764714981188035380910150706768035888671875;-0.35956743203531560393315658075152896344661712646484375]
      mask Display: e = 0.06;c1 = [120 150 230]/255;c2 = ([120 150 230]+0)/383;c3 = ([120 150 230]+128)/383;patch([0 1 1 0],[0 0 1 1],c1);patch([0 1 1 1-e 1-e 0+e],[0 0 1 1-e 0+e 0+e],c2);patch([0 0 1 1-e 0+e 0+e],[0 1 1 1-e 1-e 0+e],c3);plot([0 1 1 0 0],[0 0 1 1 0]);disp('Weights');
  "IW{1,1}(23,:)'" : Constant  Value=[-0.229645453662971232855483094681403599679470062255859375;0.7298698703765105211260788564686663448810577392578125;0.77547662452756382922558486825437285006046295166015625;0.52100721883879075324585983253200538456439971923828125;0.54468295267799626824256620238884352147579193115234375]
      mask Display: e = 0.06;c1 = [120 150 230]/255;c2 = ([120 150 230]+0)/383;c3 = ([120 150 230]+128)/383;patch([0 1 1 0],[0 0 1 1],c1);patch([0 1 1 1-e 1-e 0+e],[0 0 1 1-e 0+e 0+e],c2);patch([0 0 1 1-e 0+e 0+e],[0 1 1 1-e 1-e 0+e],c3);plot([0 1 1 0 0],[0 0 1 1 0]);disp('Weights');
  "IW{1,1}(24,:)'" : Constant  Value=[0.468031333818578587635528265309403650462627410888671875;0.9253438848612594025411226539290510118007659912109375;0.0956440096178587106923174587791436351835727691650390625;0.483121604899090228979474659354309551417827606201171875;-0.5323253718724225702629837542190216481685638427734375]
      mask Display: e = 0.06;c1 = [120 150 230]/255;c2 = ([120 150 230]+0)/383;c3 = ([120 150 230]+128)/383;patch([0 1 1 0],[0 0 1 1],c1);patch([0 1 1 1-e 1-e 0+e],[0 0 1 1-e 0+e 0+e],c2);patch([0 0 1 1-e 0+e 0+e],[0 1 1 1-e 1-e 0+e],c3);plot([0 1 1 0 0],[0 0 1 1 0]);disp('Weights');
  "IW{1,1}(25,:)'" : Constant  Value=[0.9128071754097974999098141779541037976741790771484375;-0.0175988252114218403365786258518710383214056491851806640625;-0.262039581110338370972812072068336419761180877685546875;0.6595423125647295048423757179989479482173919677734375;0.477667465501411980799417733578593470156192779541015625]
      mask Display: e = 0.06;c1 = [120 150 230]/255;c2 = ([120 150 230]+0)/383;c3 = ([120 150 230]+128)/383;patch([0 1 1 0],[0 0 1 1],c1);patch([0 1 1 1-e 1-e 0+e],[0 0 1 1-e 0+e 0+e],c2);patch([0 0 1 1-e 0+e 0+e],[0 1 1 1-e 1-e 0+e],c3);plot([0 1 1 0 0],[0 0 1 1 0]);disp('Weights');
  "IW{1,1}(26,:)'" : Constant  Value=[0.0856262262071023627640897757373750209808349609375;-0.5593797988627340345146876643411815166473388671875;-0.5833080343733063610756062189466319978237152099609375;-0.68699630649959697592521479236893355846405029296875;0.38563682766345852570566421491093933582305908203125]
      mask Display: e = 0.06;c1 = [120 150 230]/255;c2 = ([120 150 230]+0)/383;c3 = ([120 150 230]+128)/383;patch([0 1 1 0],[0 0 1 1],c1);patch([0 1 1 1-e 1-e 0+e],[0 0 1 1-e 0+e 0+e],c2);patch([0 0 1 1-e 0+e 0+e],[0 1 1 1-e 1-e 0+e],c3);plot([0 1 1 0 0],[0 0 1 1 0]);disp('Weights');
  "IW{1,1}(27,:)'" : Constant  Value=[0.0802116647187316456069083869806490838527679443359375;-0.5475827183174282186683967665885575115680694580078125;-0.118113446951352951685976222506724298000335693359375;-0.08538255889718282531930526602081954479217529296875;0.6481564267327606376767334950272925198078155517578125]
      mask Display: e = 0.06;c1 = [120 150 230]/255;c2 = ([120 150 230]+0)/383;c3 = ([120 150 230]+128)/383;patch([0 1 1 0],[0 0 1 1],c1);patch([0 1 1 1-e 1-e 0+e],[0 0 1 1-e 0+e 0+e],c2);patch([0 0 1 1-e 0+e 0+e],[0 1 1 1-e 1-e 0+e],c3);plot([0 1 1 0 0],[0 0 1 1 0]);disp('Weights');
  "IW{1,1}(28,:)'" : Constant  Value=[-0.381271651825874469121657739378861151635646820068359375;0.070084677991773369765127199570997618138790130615234375;0.903078597406235861200229919631965458393096923828125;0.244681571285711940699769684215425513684749603271484375;0.65816824679588459279244716526591219007968902587890625]
      mask Display: e = 0.06;c1 = [120 150 230]/255;c2 = ([120 150 230]+0)/383;c3 = ([120 150 230]+128)/383;patch([0 1 1 0],[0 0 1 1],c1);patch([0 1 1 1-e 1-e 0+e],[0 0 1 1-e 0+e 0+e],c2);patch([0 0 1 1-e 0+e 0+e],[0 1 1 1-e 1-e 0+e],c3);plot([0 1 1 0 0],[0 0 1 1 0]);disp('Weights');
  "IW{1,1}(29,:)'" : Constant  Value=[-0.8575308561508325766453708638437092304229736328125;0.5242194184222948027951360927545465528964996337890625;-0.7519481667039136230101803448633290827274322509765625;0.8643667100941010428272193166776560246944427490234375;-0.4132641319832159876312971391598694026470184326171875]
      mask Display: e = 0.06;c1 = [120 150 230]/255;c2 = ([120 150 230]+0)/383;c3 = ([120 150 230]+128)/383;patch([0 1 1 0],[0 0 1 1],c1);patch([0 1 1 1-e 1-e 0+e],[0 0 1 1-e 0+e 0+e],c2);patch([0 0 1 1-e 0+e 0+e],[0 1 1 1-e 1-e 0+e],c3);plot([0 1 1 0 0],[0 0 1 1 0]);disp('Weights');
  "IW{1,1}(3,:)'" : Constant  Value=[-0.3429256075093876088288880055188201367855072021484375;-0.9779398801538004004640924904379062354564666748046875;0.8392734875102263458757079206407070159912109375;0.379371862288456929146462925928062759339809417724609375;0.1676560256687527894481348766930750571191310882568359375]
      mask Display: e = 0.06;c1 = [120 150 230]/255;c2 = ([120 150 230]+0)/383;c3 = ([120 150 230]+128)/383;patch([0 1 1 0],[0 0 1 1],c1);patch([0 1 1 1-e 1-e 0+e],[0 0 1 1-e 0+e 0+e],c2);patch([0 0 1 1-e 0+e 0+e],[0 1 1 1-e 1-e 0+e],c3);plot([0 1 1 0 0],[0 0 1 1 0]);disp('Weights');
  "IW{1,1}(30,:)'" : Constant  Value=[-0.63603906566195700378330002422444522380828857421875;-0.3048656991024814022495093013276346027851104736328125;-0.058473508266086327012089896015822887420654296875;0.6701764711187025991279142544954083859920501708984375;-0.381261515154502017566073845955543220043182373046875]
      mask Display: e = 0.06;c1 = [120 150 230]/255;c2 = ([120 150 230]+0)/383;c3 = ([120 150 230]+128)/383;patch([0 1 1 0],[0 0 1 1],c1);patch([0 1 1 1-e 1-e 0+e],[0 0 1 1-e 0+e 0+e],c2);patch([0 0 1 1-e 0+e 0+e],[0 1 1 1-e 1-e 0+e],c3);plot([0 1 1 0 0],[0 0 1 1 0]);disp('Weights');
  "IW{1,1}(4,:)'" : Constant  Value=[0.74566518596807462859743509397958405315876007080078125;0.81504128868125513829312467350973747670650482177734375;-0.69158357947452209213423657274688594043254852294921875;0.970417590786032402405680841184221208095550537109375;0.7122938878608018331561879676883108913898468017578125]
      mask Display: e = 0.06;c1 = [120 150 230]/255;c2 = ([120 150 230]+0)/383;c3 = ([120 150 230]+128)/383;patch([0 1 1 0],[0 0 1 1],c1);patch([0 1 1 1-e 1-e 0+e],[0 0 1 1-e 0+e 0+e],c2);patch([0 0 1 1-e 0+e 0+e],[0 1 1 1-e 1-e 0+e],c3);plot([0 1 1 0 0],[0 0 1 1 0]);disp('Weights');
  "IW{1,1}(5,:)'" : Constant  Value=[-0.04358495983044578803156099411353352479636669158935546875;0.29969478840426500010352128811064176261425018310546875;0.441955458379438059779431569040752947330474853515625;-0.400343348413886246373039057289133779704570770263671875;-0.9080973637551303934145607854588888585567474365234375]
      mask Display: e = 0.06;c1 = [120 150 230]/255;c2 = ([120 150 230]+0)/383;c3 = ([120 150 230]+128)/383;patch([0 1 1 0],[0 0 1 1],c1);patch([0 1 1 1-e 1-e 0+e],[0 0 1 1-e 0+e 0+e],c2);patch([0 0 1 1-e 0+e 0+e],[0 1 1 1-e 1-e 0+e],c3);plot([0 1 1 0 0],[0 0 1 1 0]);disp('Weights');
  "IW{1,1}(6,:)'" : Constant  Value=[-0.1920612556581178242964824676164425909519195556640625;-0.997161883595194087348545508575625717639923095703125;0.1554777523848185349919504005811177194118499755859375;-0.7324390000111538068239269705372862517833709716796875;0.770840190969606542381598046631552278995513916015625]
      mask Display: e = 0.06;c1 = [120 150 230]/255;c2 = ([120 150 230]+0)/383;c3 = ([120 150 230]+128)/383;patch([0 1 1 0],[0 0 1 1],c1);patch([0 1 1 1-e 1-e 0+e],[0 0 1 1-e 0+e 0+e],c2);patch([0 0 1 1-e 0+e 0+e],[0 1 1 1-e 1-e 0+e],c3);plot([0 1 1 0 0],[0 0 1 1 0]);disp('Weights');
  "IW{1,1}(7,:)'" : Constant  Value=[-0.6415370471531065543757677005487494170665740966796875;-0.9392294550101645267403682737494818866252899169921875;-0.133402045581762163095618234365247189998626708984375;0.3705593688253745465743804743397049605846405029296875;-0.1845383772880364592339219598216004669666290283203125]
      mask Display: e = 0.06;c1 = [120 150 230]/255;c2 = ([120 150 230]+0)/383;c3 = ([120 150 230]+128)/383;patch([0 1 1 0],[0 0 1 1],c1);patch([0 1 1 1-e 1-e 0+e],[0 0 1 1-e 0+e 0+e],c2);patch([0 0 1 1-e 0+e 0+e],[0 1 1 1-e 1-e 0+e],c3);plot([0 1 1 0 0],[0 0 1 1 0]);disp('Weights');
  "IW{1,1}(8,:)'" : Constant  Value=[0.9364417151262116600918261610786430537700653076171875;-0.5844678305577326593578391111805103719234466552734375;0.760439078369648857602669522748328745365142822265625;0.82508941450535833173063338108477182686328887939453125;-0.928366112678612243058751118951477110385894775390625]
      mask Display: e = 0.06;c1 = [120 150 230]/255;c2 = ([120 150 230]+0)/383;c3 = ([120 150 230]+128)/383;patch([0 1 1 0],[0 0 1 1],c1);patch([0 1 1 1-e 1-e 0+e],[0 0 1 1-e 0+e 0+e],c2);patch([0 0 1 1-e 0+e 0+e],[0 1 1 1-e 1-e 0+e],c3);plot([0 1 1 0 0],[0 0 1 1 0]);disp('Weights');
  "IW{1,1}(9,:)'" : Constant  Value=[-0.1850570281869012012609942985363886691629886627197265625;-0.090036213787947183551096941300784237682819366455078125;-0.2138649950013847556018475870587280951440334320068359375;0.2217666609154813894821955955194425769150257110595703125;0.492316969493460099283055342311854474246501922607421875]
      mask Display: e = 0.06;c1 = [120 150 230]/255;c2 = ([120 150 230]+0)/383;c3 = ([120 150 230]+128)/383;patch([0 1 1 0],[0 0 1 1],c1);patch([0 1 1 1-e 1-e 0+e],[0 0 1 1-e 0+e 0+e],c2);patch([0 0 1 1-e 0+e 0+e],[0 1 1 1-e 1-e 0+e],c3);plot([0 1 1 0 0],[0 0 1 1 0]);disp('Weights');
  Mux : Mux  Inputs=30
      mask Display: e = 0.06;c1 = [120 150 230]/255;c2 = ([120 150 230]+0)/383;c3 = ([120 150 230]+128)/383;patch([0 1 1 0],[0 0 1 1],c1);patch([0 1 1 1-e 1-e 0+e],[0 0 1 1-e 0+e 0+e],c2);patch([0 0 1 1-e 0+e 0+e],[0 1 1 1-e 1-e 0+e],c3);plot([0 1 1 0 0],[0 0 1 1 0]);disp('Mux');
  dotprod{1..30} (30 alike) : neural/Weight Functions/dotprod
  "iz{1,1}" : Outport
      mask Display: e = 0.06;c1 = [120 230 180]/255;c2 = ([120 230 180]+0)/(256+128);c3 = ([120 230 180]+128)/(256+128);patch([0 1 1 0],[0 0 1 1],c1);patch([0 1 1 1-e 1-e 0+e],[0 0 1 1-e 0+e 0+e],c2);patch([0 0 1 1-e 0+e 0+e],[0 1 1 1-e 1-e 0+e],c3);plot([0 1 1 0 0],[0 0 1 1 0]);
  wires:
  Mux/1 -> "iz{1,1}"/1
  dotprod30/1 -> Mux/30
  "IW{1,1}(30,:)'"/1 -> dotprod30/1
  dotprod29/1 -> Mux/29
  "IW{1,1}(29,:)'"/1 -> dotprod29/1
  dotprod28/1 -> Mux/28
  "IW{1,1}(28,:)'"/1 -> dotprod28/1
  dotprod27/1 -> Mux/27
  "IW{1,1}(27,:)'"/1 -> dotprod27/1
  dotprod26/1 -> Mux/26
  "IW{1,1}(26,:)'"/1 -> dotprod26/1
  dotprod25/1 -> Mux/25
  "IW{1,1}(25,:)'"/1 -> dotprod25/1
  dotprod24/1 -> Mux/24
  "IW{1,1}(24,:)'"/1 -> dotprod24/1
  dotprod23/1 -> Mux/23
  "IW{1,1}(23,:)'"/1 -> dotprod23/1
  dotprod22/1 -> Mux/22
  "IW{1,1}(22,:)'"/1 -> dotprod22/1
  dotprod21/1 -> Mux/21
  "IW{1,1}(21,:)'"/1 -> dotprod21/1
  dotprod20/1 -> Mux/20
  "IW{1,1}(20,:)'"/1 -> dotprod20/1
  dotprod19/1 -> Mux/19
  "IW{1,1}(19,:)'"/1 -> dotprod19/1
  dotprod18/1 -> Mux/18
  "IW{1,1}(18,:)'"/1 -> dotprod18/1
  dotprod17/1 -> Mux/17
  "IW{1,1}(17,:)'"/1 -> dotprod17/1
  dotprod16/1 -> Mux/16
  "IW{1,1}(16,:)'"/1 -> dotprod16/1
  dotprod15/1 -> Mux/15
  "IW{1,1}(15,:)'"/1 -> dotprod15/1
  dotprod14/1 -> Mux/14
  "IW{1,1}(14,:)'"/1 -> dotprod14/1
  dotprod13/1 -> Mux/13
  "IW{1,1}(13,:)'"/1 -> dotprod13/1
  dotprod12/1 -> Mux/12
  "IW{1,1}(12,:)'"/1 -> dotprod12/1
  dotprod11/1 -> Mux/11
  "IW{1,1}(11,:)'"/1 -> dotprod11/1
  dotprod10/1 -> Mux/10
  "IW{1,1}(10,:)'"/1 -> dotprod10/1
  dotprod9/1 -> Mux/9
  "IW{1,1}(9,:)'"/1 -> dotprod9/1
  dotprod8/1 -> Mux/8
  "IW{1,1}(8,:)'"/1 -> dotprod8/1
  dotprod7/1 -> Mux/7
  "IW{1,1}(7,:)'"/1 -> dotprod7/1
  dotprod6/1 -> Mux/6
  "IW{1,1}(6,:)'"/1 -> dotprod6/1
  dotprod5/1 -> Mux/5
  "IW{1,1}(5,:)'"/1 -> dotprod5/1
  dotprod4/1 -> Mux/4
  "IW{1,1}(4,:)'"/1 -> dotprod4/1
  dotprod3/1 -> Mux/3
  "IW{1,1}(3,:)'"/1 -> dotprod3/1
  dotprod2/1 -> Mux/2
  "IW{1,1}(2,:)'"/1 -> dotprod2/1
  dotprod1/1 -> Mux/1
  "pd{1,1}"/1 -> dotprod30/2, dotprod29/2, dotprod28/2, dotprod27/2, dotprod26/2, dotprod25/2, dotprod24/2, dotprod23/2, dotprod22/2, dotprod21/2, dotprod20/2, dotprod19/2, dotprod18/2, dotprod17/2, dotprod16/2, dotprod15/2, dotprod14/2, dotprod13/2, dotprod12/2, dotprod11/2, dotprod10/2, dotprod9/2, dotprod8/2, dotprod7/2, dotprod6/2, dotprod5/2, dotprod4/2, dotprod3/2, dotprod2/2, dotprod1/2
  "IW{1,1}(1,:)'"/1 -> dotprod1/1

== system ACC4_FFNN_trainoss_30_30_30_ep_100_Nor_20250528/Feed-Forward Neural Network/Layer 2/Delays 1 ==
  "p{2}" : Inport  PortDimensions=30
      mask Display: e = 0.06;c1 = [120 230 180]/255;c2 = ([120 230 180]+0)/(256+128);c3 = ([120 230 180]+128)/(256+128);patch([0 1 1 0],[0 0 1 1],c1);patch([0 1 1 1-e 1-e 0+e],[0 0 1 1-e 0+e 0+e],c2);patch([0 0 1 1-e 0+e 0+e],[0 1 1 1-e 1-e 0+e],c3);plot([0 1 1 0 0],[0 0 1 1 0]);
  mux : Mux  Inputs=1
      mask Display: e = 0.06;c1 = [120 150 230]/255;c2 = ([120 150 230]+0)/383;c3 = ([120 150 230]+128)/383;patch([0 1 1 0],[0 0 1 1],c1);patch([0 1 1 1-e 1-e 0+e],[0 0 1 1-e 0+e 0+e],c2);patch([0 0 1 1-e 0+e 0+e],[0 1 1 1-e 1-e 0+e],c3);plot([0 1 1 0 0],[0 0 1 1 0]);disp('Mux')
  "pd{2,1}" : Outport
      mask Display: e = 0.06;c1 = [120 230 180]/255;c2 = ([120 230 180]+0)/(256+128);c3 = ([120 230 180]+128)/(256+128);patch([0 1 1 0],[0 0 1 1],c1);patch([0 1 1 1-e 1-e 0+e],[0 0 1 1-e 0+e 0+e],c2);patch([0 0 1 1-e 0+e 0+e],[0 1 1 1-e 1-e 0+e],c3);plot([0 1 1 0 0],[0 0 1 1 0]);
  wires:
  mux/1 -> "pd{2,1}"/1
  "p{2}"/1 -> mux/1
